simulink model "Exp01"  (R2024b)
settings: Solver=VariableStepAuto  StartTime=0.0  StopTime=0.02  RelTol=1e-3
libraries: spsRMSLib x4, eePowerMeasurement x3, spsVoltageMeasurementLib x3, spsSeriesRLCBranchLib x2, spsACVoltageSourceLib x1, spsCurrentMeasurementLib x1, sps_lib x1
settings Model: Creator=HP  LastModifiedBy=HP

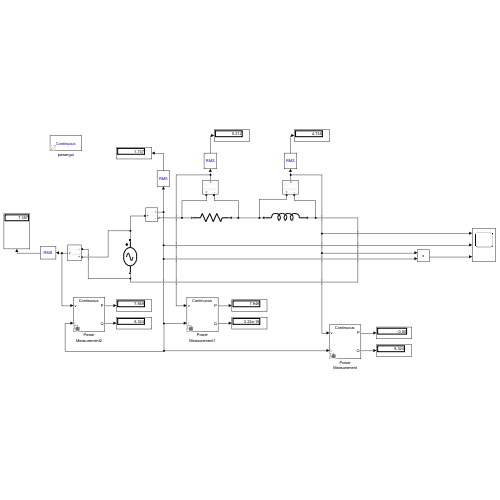
[thumbnail: Simulink's stored preview of the top-level diagram]
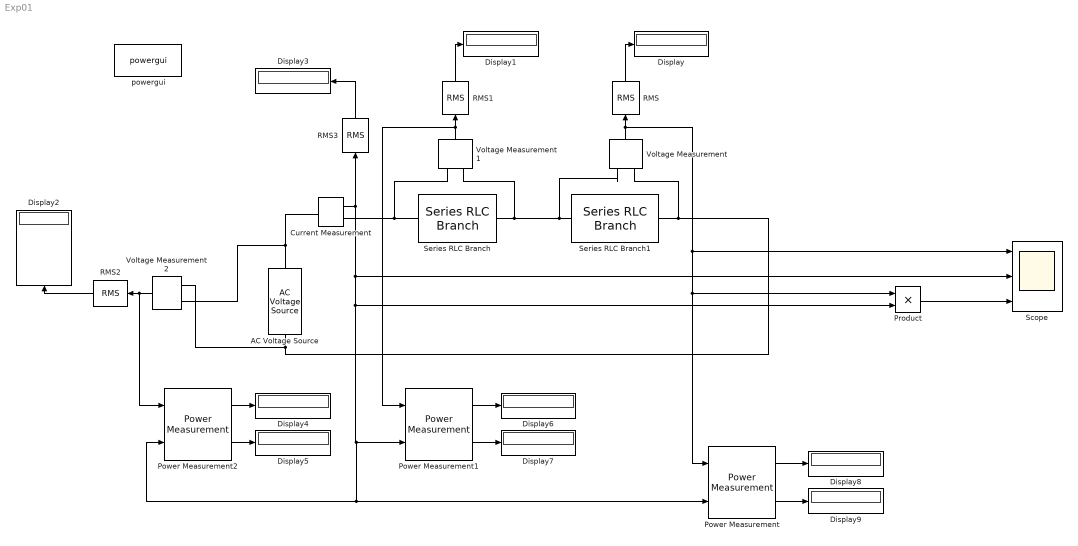
== system Exp01 ==
  AC Voltage Source : spsACVoltageSourceLib/AC Voltage Source  Amplitude=10  Phase=0  Frequency=50  SampleTime=0  Measurements=None  BusType=swing  Pref=10e3  Qref=0  Qmin=-inf  Qmax=+inf
  Current Measurement : spsCurrentMeasurementLib/Current Measurement  PhasorSimulation=off  OutputType=Complex  PSBequivalent=0
  Display{,1..9} (10 alike) : Display
      Display8 settings: Format=bank
  Power Measurement : eePowerMeasurement/Power Measurement  LabelModeActiveChoice=Continuous  F=50  K=[1]  Ts=0
  Power Measurement1 : eePowerMeasurement/Power Measurement  LabelModeActiveChoice=Continuous  F=50  K=[1]  Ts=0
  Power Measurement2 : eePowerMeasurement/Power Measurement  LabelModeActiveChoice=Continuous  F=50  K=[1]  Ts=0
  Product : Product
  RMS{,1..3} (4 alike) : spsRMSLib/RMS  TrueRMS=on  Freq=60  RMSInit=120  Ts=0
  Scope : Scope  NumInputPorts=3
  Series RLC Branch : spsSeriesRLCBranchLib/Series RLC Branch  LConnTagsString=__new0  RConnTagsString=__new0  BranchType=R  Resistance=3  Inductance=1e-3  SetiL0=off  InitialCurrent=0  Capacitance=1e-6  Setx0=off  InitialVoltage=0  Measurements=None
  Series RLC Branch1 : spsSeriesRLCBranchLib/Series RLC Branch  LConnTagsString=__new0  RConnTagsString=__new0  BranchType=L  Resistance=1  Inductance=1e-2  SetiL0=off  InitialCurrent=0  Capacitance=1e-6  Setx0=off  InitialVoltage=0  Measurements=None
  Voltage Measurement : spsVoltageMeasurementLib/Voltage Measurement  PhasorSimulation=off  OutputType=Complex  PSBequivalent=0
  Voltage Measurement1 : spsVoltageMeasurementLib/Voltage Measurement  PhasorSimulation=off  OutputType=Complex  PSBequivalent=0
  Voltage Measurement2 : spsVoltageMeasurementLib/Voltage Measurement  PhasorSimulation=off  OutputType=Complex  PSBequivalent=0
  powergui : sps_lib/powergui  Priority=1  SimulationMode=Continuous  SampleTime=50e-6  frequency=60  Iterations=50  frequencyindice=50  Pbase=100e6  ErrMax=1e-4  UnitsV=kV  UnitsW=MW  buscounter=0  FunctionMessages=off  echomessages=off  EnableUseOfTLC=off  CurrentSourceSwitches=off  DisableSnubberDevices=off  DisableRonSwitches=off  DisableVfSwitches=off  DisplayEquations=off  AutomaticDiscreteSolvers=off  SolverType=Tustin/Backward Euler (TBE)  Interpol=off  ExternalGateDelay=off  methode=off  Ts=100  x0status=blocks  SPID=on  SwTol=0  HookPort=off  NonlinearTolerance=1e-4  nMaxIteration=100  ContinueOnMaxIteration=off  RestoreLinks=warning  ResistiveCurrentMeasurement=off  Frange=[0:2:500]  Ylog=off  Xlog=on  ShowGrid=off  save=off  variable=ZData  structure=0  ZoomFFT=off  StartTime=0.0  cycles=1  DisplayStyle=1  fundamental=60  FreqAxis=off  MaxFrequency=1000  frequencyindicesteady=1  RmsSteady=1  display=off
  wires:
  Voltage Measurement/1 -> Scope/1, Product/1, Power Measurement/1, RMS/1
  RMS/1 -> Display/1
  RMS1/1 -> Display1/1
  Voltage Measurement1/1 -> Power Measurement1/1, RMS1/1
  RMS2/1 -> Display2/1
  Voltage Measurement2/1 -> Power Measurement2/1, RMS2/1
  Current Measurement/1 -> RMS3/1, Scope/2, Product/2, Power Measurement2/2, Power Measurement/2, Power Measurement1/2
  RMS3/1 -> Display3/1
  Power Measurement2/2 -> Display5/1
  Power Measurement2/1 -> Display4/1
  Power Measurement1/1 -> Display6/1
  Power Measurement1/2 -> Display7/1
  Power Measurement/1 -> Display8/1
  Power Measurement/2 -> Display9/1
  Product/1 -> Scope/3
  connections:
  Series RLC Branch1/LConn1 -- Voltage Measurement1/LConn2 -- Series RLC Branch/RConn1 -- Voltage Measurement/LConn1
  AC Voltage Source/LConn1 -- Voltage Measurement2/LConn2 -- Voltage Measurement/LConn2 -- Series RLC Branch1/RConn1
  AC Voltage Source/RConn1 -- Voltage Measurement2/LConn1 -- Current Measurement/LConn1
  Current Measurement/RConn1 -- Voltage Measurement1/LConn1 -- Series RLC Branch/LConn1
